simulink model "Rebuilt_Shooter_Test"  (R2023b)
settings: Solver=VariableStepAuto  StartTime=0.0  StopTime=20  MaxStep=0.02  RelTol=1e-3
values from neighbouring files (symbols this model uses):
  Blue_Hub_X = 182.11*0.0254    (= 4.625594)    [Rebuilt_Shooter_Test_data.m]
  Blue_Hub_Y = 158.84*0.0254    (= 4.034536)    [Rebuilt_Shooter_Test_data.m]
settings Model: Creator=ander  LastModifiedBy=ander

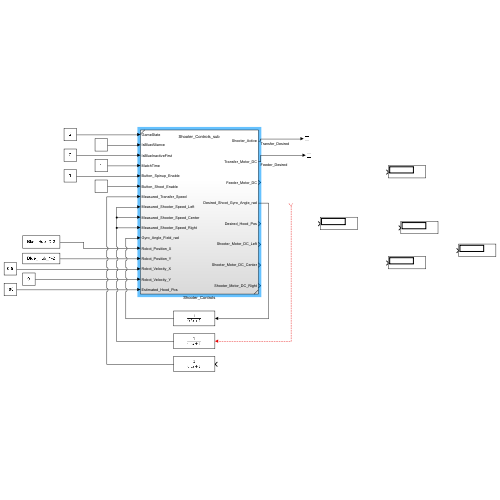
[thumbnail: Simulink's stored preview of the top-level diagram]
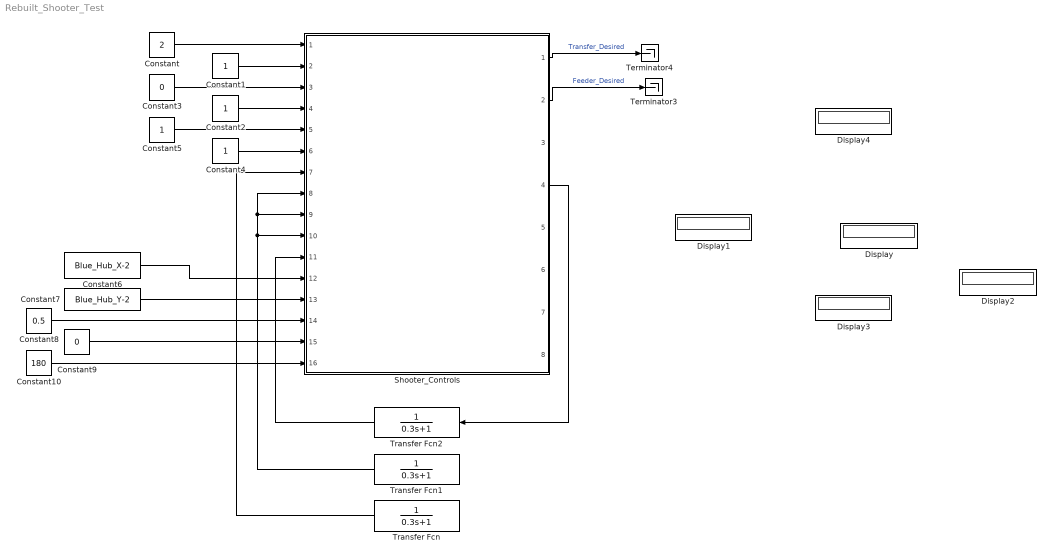
== system Rebuilt_Shooter_Test ==
  Constant : Constant  Value=2
  Constant1 : Constant  OutDataTypeStr=boolean
  Constant10 : Constant  Value=180
  Constant2 : Constant
  Constant3 : Constant  Value=0  OutDataTypeStr=boolean
  Constant4 : Constant
  Constant5 : Constant
  Constant6 : Constant  Value=Blue_Hub_X-2
  Constant7 : Constant  Value=Blue_Hub_Y-2
  Constant8 : Constant  Value=0.5
  Constant9 : Constant  Value=0
  Display{,1..4} (5 alike) : Display
  Shooter_Controls : Subsystem  ReferencedSubsystem=Shooter_Controls_sub
  Terminator3 : Terminator
  Terminator4 : Terminator
  Transfer Fcn : TransferFcn  Denominator=[0.3 1]
  Transfer Fcn1 : TransferFcn  Denominator=[0.3 1]
  Transfer Fcn2 : TransferFcn  Denominator=[0.3 1]
  wires:
  Shooter_Controls/2 -> Terminator3/1  "Feeder_Desired"
  Shooter_Controls/1 -> Terminator4/1  "Transfer_Desired"
  Transfer Fcn/1 -> Shooter_Controls/7
  Transfer Fcn1/1 -> Shooter_Controls/8, Shooter_Controls/9, Shooter_Controls/10
  Transfer Fcn2/1 -> Shooter_Controls/11
  Constant/1 -> Shooter_Controls/1
  Constant1/1 -> Shooter_Controls/2
  Constant3/1 -> Shooter_Controls/3
  Constant2/1 -> Shooter_Controls/4
  Constant5/1 -> Shooter_Controls/5
  Constant4/1 -> Shooter_Controls/6
  Constant6/1 -> Shooter_Controls/12
  Constant7/1 -> Shooter_Controls/13
  Constant8/1 -> Shooter_Controls/14
  Constant9/1 -> Shooter_Controls/15
  Constant10/1 -> Shooter_Controls/16
  Shooter_Controls/4 -> Transfer Fcn2/1
  ? -> Transfer Fcn1/1
